simulink model "IRMessung1"  (R2026b)
settings: Solver=FixedStepDiscrete  StopTime=30  FixedStep=0.01  EnableMultiTasking=on
model workspace (MAT data in the model file):
  PAR_SenIr_Abtast_f64 : Simulink.Parameter (value not decoded)
  PAR_SenIr_URef_f32 : Simulink.Parameter (value not decoded)
symbols that are objects in the model workspace (value not decoded): PAR_SenIr_Abtast_f64, PAR_SenIr_URef_f32
libraries: arduinolib x1
settings Model: SILPILModeSetting=veronly
settings SolverCC: AutoInsertRateTranBlk=on
settings OptimizationCC: DifferentSizesBufferReuse=on  EfficientTunableParamExpr=on  EnhancedBackFolding=on  MaxStackSize=64  OptimizationCustomize=off  OptimizeBlockOrder=speed  PassReuseOutputArgsAs=Individual arguments  RemoveInternalMemoryZeroInit=on  RemoveRootLevelIOMemoryZeroInit=on
settings DebuggingCC: ParameterTunabilityLossMsg=error
settings HardwareCC: ProdHWDeviceType=Atmel->AVR  ProdLargestAtomicFloat=None
settings SFSimCC: MATLABDynamicMemAlloc=off
settings RTWCC: BuildConfiguration=Faster Runs  Description=Embedded Coder  HardwareBoard=Arduino Uno  SystemTargetFile=ert.tlc  TLCOptions=-aInlineSetEventsForThisBaseRateFcn=TLC_FALSE -aSuppressMultiTaskScheduler=TLC_FALSE -aRateBasedStepFcn=1  TemplateMakefile=ert_default_tmf  Toolchain=Arduino AVR
settings CodeAppCC: ForceParamTrailComments=on  IgnoreCustomStorageClasses=off  InsertBlockDesc=on  OperatorAnnotations=on  SFDataObjDesc=on  SimulinkDataObjDesc=on
settings ERTTargetCC: CombineSignalStateStructs=on  ExtModeAutomaticAllocSize=off  ExtModeIntrfLevel=Level2 - Open  ExtModeMexFile=ext_xcp  ExtModeStaticAlloc=on  SupportContinuousTime=on  SupportVariableSizeSignals=on

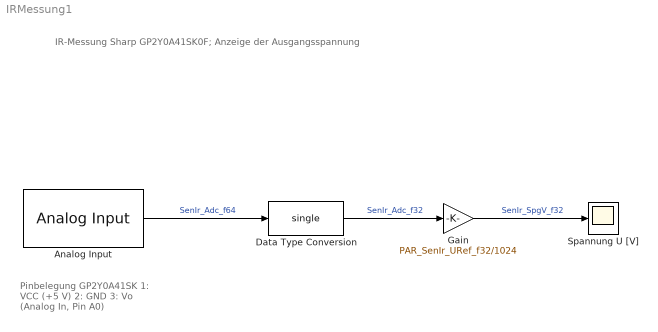
== system IRMessung1 ==
  note: Pinbelegung GP2Y0A41SK
      | 1: VCC (+5 V)
      | 2: GND
      | 3: Vo (Analog In, Pin A0)
  note: IR-Messung Sharp GP2Y0A41SK0F; Anzeige der Ausgangsspannung
  Analog Input : arduinolib/Analog Input  pinNumber=0  ReadResultsOnly=off  ConversionTriggerSource=Software  ExternalTriggerType=uint32( 0 )  OutputDataType=uint16  EnableConversionCompleteNotify=off  EnableOuputStatus=off  SampleTime=PAR_SenIr_Abtast_f64  blockPlatform=arduino
  Data Type Conversion : DataTypeConversion  OutDataTypeStr=single  SaturateOnIntegerOverflow=off  RndMeth=Floor
  Gain : Gain  Gain=PAR_SenIr_URef_f32/1024
  Spannung U [V] : Scope
      settings: ActiveDisplayYMinimum=-0.365786542970141  ActiveDisplayYMaximum=5.4230944032384443
  wires:
  Analog Input/1 -> Data Type Conversion/1  "SenIr_Adc_f64"
  Data Type Conversion/1 -> Gain/1  "SenIr_Adc_f32"
  Gain/1 -> Spannung U [V]/1  "SenIr_SpgV_f32"
